simulink model "mars_zemzev"  (R2025a)
settings: Solver=VariableStepAuto  StartTime=0.0  StopTime=90  RelTol=1e-3
undefined symbols (not defined in the file or in its folder): kr
settings Model: Creator=dom  LastModifiedBy=dom

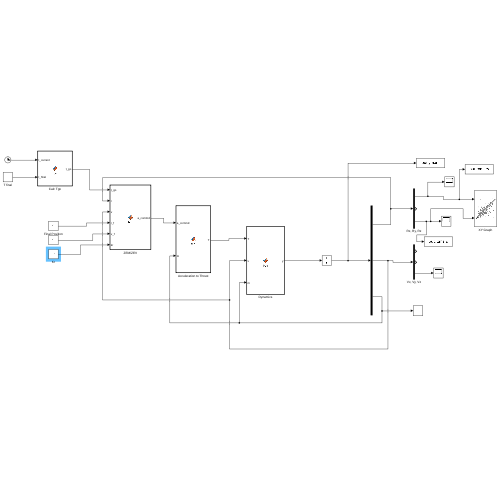
[thumbnail: Simulink's stored preview of the top-level diagram]
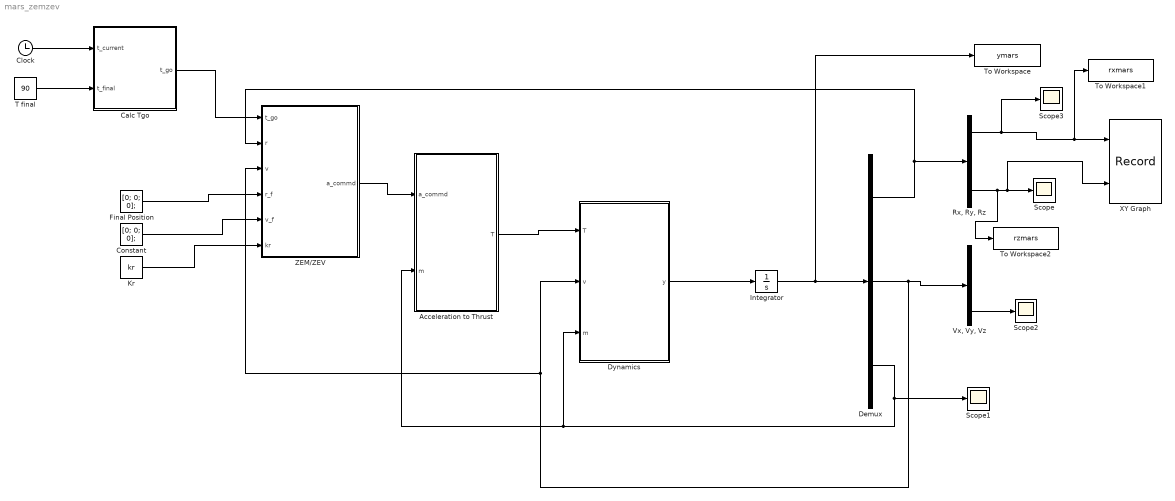
== system mars_zemzev ==
  Acceleration to Thrust : MATLAB Function  TreatAsAtomicUnit=on
  Calc Tgo : MATLAB Function  TreatAsAtomicUnit=on
  Clock : Clock
  Constant : Constant  Value=[0; 0; 0];
  Demux : Demux  Outputs=[3 3 1]
  Dynamics : MATLAB Function  TreatAsAtomicUnit=on
  Final Position : Constant  Value=[0; 0; 0];
  Integrator : Integrator  InitialCondition=[1500; 0; 3000; 100; 0; -75; 1905];
  Kr : Constant  Value=kr
  "Rx, Ry, Rz" : Demux  Outputs=3
  Scope{,1..3} (4 alike) : Scope
      Scope settings: ActiveDisplayYMinimum=-2531.5676765984049  ActiveDisplayYMaximum=4380.1207422296966
      Scope1 settings: ActiveDisplayYMinimum=1542.3699052525453  ActiveDisplayYMaximum=1945.2922327497172
      Scope2 settings: ActiveDisplayYMinimum=-1  ActiveDisplayYMaximum=1  DataLoggingVariableName=ScopeData2
      Scope3 settings: ActiveDisplayYMinimum=-381.29193428417022  ActiveDisplayYMaximum=3431.6268392693009  DataLoggingVariableName=ScopeData3
  T final : Constant  Value=90
  To Workspace : ToWorkspace  VariableName=ymars  SaveFormat=Timeseries  SampleTime=-1
  To Workspace1 : ToWorkspace  VariableName=rxmars  SaveFormat=Timeseries  SampleTime=-1
  To Workspace2 : ToWorkspace  VariableName=rzmars  SaveFormat=Timeseries  SampleTime=-1
  "Vx, Vy, Vz" : Demux  Outputs=3
  XY Graph : Record  NumPorts=2.0  FileSettingsInternal="{\"entries\":[{\"content\":{\"excelSettings\":{\"content\":{},\"type\":\"Streamout.ExcelSettings\"},\"parquetSettings\":{\"content\":{},\"type\":\"Streamout.ParquetSettings\"}},\"type\":\"Streamout.FileSettingStorage\",\"uuid\":\"\"}],\"packageUris\":[\"http:\\/\\/schema.mathworks.com\\/mf0\\/streamout_blocks\\/R2020a\"],\"version\":\"1.0\"}"  FrameSettings=[0, 0]  Layout=[1 1]  SignalsInternal="{\"entries\":[{\"content\":{\"signals\":[{\"content\":{\"blockPath\":[],\"dimensions\":[1,1],\"domain\":\"\",\"lineColor\":\"#a2142f\",\"plots\":[ 1 ],\"port\":1,\"signalID\":1,\"signalName\":\"Rx, Ry, Rz:1\"},\"type\":\"RecordBlkView.Signal\",\"uuid\":\"\"},{\"content\":{\"blockPath\":[],\"dimensions\":[1,1],\"domain\":\"\",\"lineColor\":\"#139fff\",\"plots\":[ 1 ],\"port\":2,\"signalID\":2,\"signalName\":\"Rx, Ry, Rz:3\"},\"type\":\"RecordBlkView.Signal\",\"uuid\":\"\"}]},\"type\":\"RecordBlkView.InputSignals\",\"uuid\":\"\"}],\"packageUris\":[\"http:\\/\\/schema.mathworks.com\\/mf0\\/streamout_blocks\\/R2020a\"],\"version\":\"1.0\"}"  VisualizationBindings="{\"xyplotplugin\":{\"info\":[{\"series\":[{\"bindingParametersList\":[{\"parameter\":\"X-Axis\",\"signalID\":1,\"signalName\":\"Rx, Ry, Rz:1\"},{\"parameter\":\"Y-Axis\",\"signalID\":2,\"signalName\":\"Rx, Ry, Rz:3\"}],\"seriesID\":0}],\"subplotID\":1}]}}"  CompatibilityTag=XY
  ZEM/ZEV : MATLAB Function  TreatAsAtomicUnit=on
  wires:
  T final/1 -> Calc Tgo/2(t_final)
  Clock/1 -> Calc Tgo/1(t_current)
  Calc Tgo/1(t_go) -> ZEM/ZEV/1(t_go)
  Final Position/1 -> ZEM/ZEV/4(r_f)
  Constant/1 -> ZEM/ZEV/5(v_f)
  ZEM/ZEV/1(a_commd) -> Acceleration to Thrust/1(a_commd)
  Acceleration to Thrust/1(T) -> Dynamics/1(T)
  Dynamics/1(y) -> Integrator/1
  Integrator/1 -> To Workspace/1, Demux/1
  Demux/1 -> "Rx, Ry, Rz"/1, ZEM/ZEV/2(r)
  Demux/2 -> ZEM/ZEV/3(v), Dynamics/2(v), "Vx, Vy, Vz"/1
  Demux/3 -> Scope1/1, Acceleration to Thrust/2(m), Dynamics/3(m)
  "Rx, Ry, Rz"/3 -> To Workspace2/1, XY Graph/2, Scope/1
  "Rx, Ry, Rz"/1 -> Scope3/1, To Workspace1/1, XY Graph/1
  "Vx, Vy, Vz"/3 -> Scope2/1
  Kr/1 -> ZEM/ZEV/6(kr)

== matlab function mars_zemzev/ZEM//ZEV ==
  data: t_go input; a_commd output; r input; v input; r_f input; v_f input; kr input
function a_commd = fcn(t_go, r, v, r_f, v_f, kr)
g=[0; 0; -3.7114];


switch kr
    case 6
        a_commd=(kr/t_go^2)*(r_f-(r+t_go*v))+2/t_go*(1-kr/3)*(v_f-v);
    case 12
        a_commd=(kr/t_go^2)*(r_f-(r+t_go*v))+(2/t_go)*(1-kr/3)*(v_f-v)-(kr/6)*g;
    case 15
        ZEM= r_f-(r+t_go*v+0.5*g*t_go^2);
        ZEV = v_f - (v+g*t_go);
        a_commd= (kr/t_go^2)*ZEM - (8/t_go)*ZEV - 3*g;
    otherwise
        a_commd=zeros(3,1);

end

== matlab function mars_zemzev/Calc Tgo ==
  data: t_current input; t_go output; t_final input
function t_go = fcn(t_current, t_final)

t_go = 1.001*t_final - t_current;

== matlab function mars_zemzev/Acceleration to Thrust ==
  data: a_commd input; T output; m input
function T = fcn(a_commd, m)

n=6;
Fmax=3100;
phi=deg2rad(10);

% set minimum thrust value in
T_min = 0.3*n*Fmax*cos(phi);
% set max T value
T_max = 0.8*n*Fmax*cos(phi);

a = a_commd;

% adjust thrust value if T falls outside Tmin/Tmax
if norm(a) >= T_max/m
    a=a/norm(a)*T_max/m;
elseif norm(a)<= T_min/m && norm(a)~=0
    a=a/norm(a)*T_min/m;
end

T=a*m;

== matlab function mars_zemzev/Dynamics ==
  data: T input; v input; y output; m input
function y = fcn(T, v, m)

% set constants
% gravity
g = [0; 0; -3.7114];
% intial gravity
g_0 = 9.8;

I_sp = 225;

c=I_sp*g_0;
phi=deg2rad(10);

% dynamics equations
r_dot=v;
v_dot=g+(T/m);
m_dot=-(norm(T)/cos(phi))/(I_sp*g_0);



y = [r_dot; v_dot; m_dot];
